simulink model "Partie6_RRC"  (R2026b)
settings: Solver=FixedStepDiscrete  StopTime=Nbits*Tb  FixedStep=Tf
undefined symbols (not defined in the file): D_ech, graine, graine_bruit, h_rx, h_tx, p1, Tb, Te, variance_bruit_p6
libraries: simulink x2, dspsigops x1
settings Model: Creator=WORLD COMPUTERS  LastModifiedBy=WORLD COMPUTERS

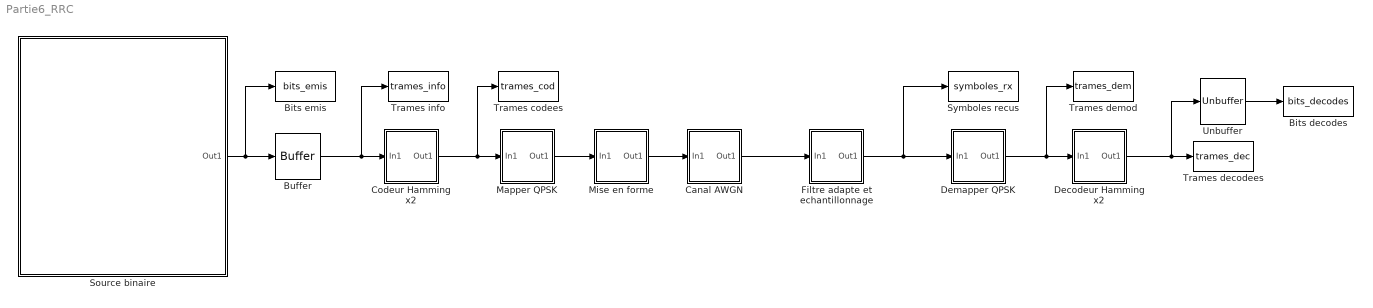
== system Partie6_RRC ==
  Bits decodes : ToWorkspace  VariableName=bits_decodes  SampleTime=-1
  Bits emis : ToWorkspace  VariableName=bits_emis  SampleTime=-1
  Buffer : Buffer  N=8
  Canal AWGN : Subsystem
  Codeur Hamming x2 : Subsystem
  Decodeur Hamming x2 : Subsystem
  Demapper QPSK : Subsystem
  Filtre adapte et echantillonnage : Subsystem
  Mapper QPSK : Subsystem
  Mise en forme : Subsystem
  Source binaire : Subsystem
  Symboles recus : ToWorkspace  VariableName=symboles_rx  SampleTime=-1
  Trames codees : ToWorkspace  VariableName=trames_cod  SampleTime=-1
  Trames decodees : ToWorkspace  VariableName=trames_dec  SampleTime=-1
  Trames demod : ToWorkspace  VariableName=trames_dem  SampleTime=-1
  Trames info : ToWorkspace  VariableName=trames_info  SampleTime=-1
  Unbuffer : Unbuffer
  wires:
  Source binaire/1(Out1) -> Buffer/1, Bits emis/1
  Demapper QPSK/1(Out1) -> Trames demod/1, Decodeur Hamming x2/1(In1)
  Buffer/1 -> Codeur Hamming x2/1(In1), Trames info/1
  Codeur Hamming x2/1(Out1) -> Mapper QPSK/1(In1), Trames codees/1
  Mapper QPSK/1(Out1) -> Mise en forme/1(In1)
  Mise en forme/1(Out1) -> Canal AWGN/1(In1)
  Filtre adapte et echantillonnage/1(Out1) -> Demapper QPSK/1(In1), Symboles recus/1
  Canal AWGN/1(Out1) -> Filtre adapte et echantillonnage/1(In1)
  Decodeur Hamming x2/1(Out1) -> Unbuffer/1, Trames decodees/1
  Unbuffer/1 -> Bits decodes/1

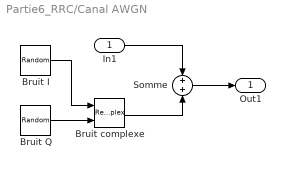
== system Partie6_RRC/Canal AWGN ==
  In1 : Inport
  Bruit I : RandomNumber  Variance=variance_bruit_p6  Seed=graine_bruit  SampleTime=Te
  Bruit Q : RandomNumber  Variance=variance_bruit_p6  Seed=graine_bruit+100  SampleTime=Te
  Bruit complexe : RealImagToComplex
  Somme : Sum
  Out1 : Outport
  wires:
  Bruit I/1 -> Bruit complexe/1
  Bruit complexe/1 -> Somme/2
  In1/1 -> Somme/1
  Bruit Q/1 -> Bruit complexe/2
  Somme/1 -> Out1/1

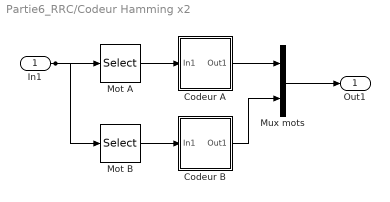
== system Partie6_RRC/Codeur Hamming x2 ==
  In1 : Inport
  Codeur A : Subsystem
  Codeur B : Subsystem
  Mot A : Selector  InputPortWidth=8  IndexOptions=Index vector (dialog)  Indices=[1 2 3 4]  OutputSizes=1
  Mot B : Selector  InputPortWidth=8  IndexOptions=Index vector (dialog)  Indices=[5 6 7 8]  OutputSizes=1
  Mux mots : Mux  Inputs=2
  Out1 : Outport
  wires:
  Mot B/1 -> Codeur B/1(In1)
  In1/1 -> Mot A/1, Mot B/1
  Codeur A/1(Out1) -> Mux mots/1
  Mot A/1 -> Codeur A/1(In1)
  Codeur B/1(Out1) -> Mux mots/2
  Mux mots/1 -> Out1/1

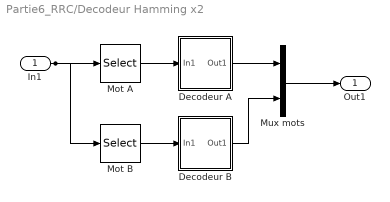
== system Partie6_RRC/Decodeur Hamming x2 ==
  In1 : Inport
  Decodeur A : Subsystem
  Decodeur B : Subsystem
  Mot A : Selector  InputPortWidth=14  IndexOptions=Index vector (dialog)  Indices=[1 2 3 4 5 6 7]  OutputSizes=1
  Mot B : Selector  InputPortWidth=14  IndexOptions=Index vector (dialog)  Indices=[8 9 10 11 12 13 14]  OutputSizes=1
  Mux mots : Mux  Inputs=2
  Out1 : Outport
  wires:
  Mot B/1 -> Decodeur B/1(In1)
  In1/1 -> Mot A/1, Mot B/1
  Mot A/1 -> Decodeur A/1(In1)
  Decodeur A/1(Out1) -> Mux mots/1
  Decodeur B/1(Out1) -> Mux mots/2
  Mux mots/1 -> Out1/1

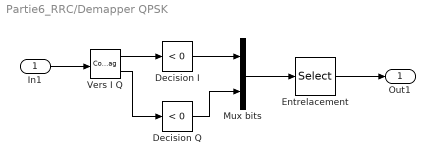
== system Partie6_RRC/Demapper QPSK ==
  In1 : Inport
  Decision I : simulink/Logic and Bit Operations/Compare To Constant  relop=<  const=0  OutDataTypeStr=boolean
  Decision Q : simulink/Logic and Bit Operations/Compare To Constant  relop=<  const=0  OutDataTypeStr=boolean
  Entrelacement : Selector  InputPortWidth=14  IndexOptions=Index vector (dialog)  Indices="[1   8   2   9   3  10   4  11   5  12   6  13   7  14]"  OutputSizes=1
  Mux bits : Mux  Inputs=2
  Vers I Q : ComplexToRealImag
  Out1 : Outport
  wires:
  Entrelacement/1 -> Out1/1
  In1/1 -> Vers I Q/1
  Mux bits/1 -> Entrelacement/1
  Decision Q/1 -> Mux bits/2
  Vers I Q/1 -> Decision I/1
  Vers I Q/2 -> Decision Q/1
  Decision I/1 -> Mux bits/1

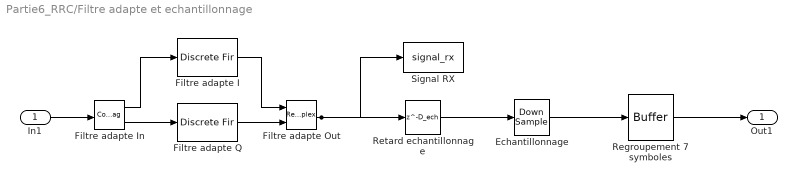
== system Partie6_RRC/Filtre adapte et echantillonnage ==
  In1 : Inport
  Echantillonnage : DownSample  DownsamplingFactor=L  RateOptions=Allow multirate processing  AllowArbitraryFixedInput=on
  Filtre adapte I : DiscreteFir  Coefficients=h_rx
  Filtre adapte In : ComplexToRealImag
  Filtre adapte Out : RealImagToComplex
  Filtre adapte Q : DiscreteFir  Coefficients=h_rx
  Regroupement 7 symboles : Buffer  N=7
  Retard echantillonnage : Delay  DelayLength=D_ech  InitialCondition=0
  Signal RX : ToWorkspace  VariableName=signal_rx  SampleTime=-1
  Out1 : Outport
  wires:
  Echantillonnage/1 -> Regroupement 7 symboles/1
  Retard echantillonnage/1 -> Echantillonnage/1
  Filtre adapte Out/1 -> Retard echantillonnage/1, Signal RX/1
  In1/1 -> Filtre adapte In/1
  Filtre adapte Q/1 -> Filtre adapte Out/2
  Filtre adapte I/1 -> Filtre adapte Out/1
  Filtre adapte In/2 -> Filtre adapte Q/1
  Filtre adapte In/1 -> Filtre adapte I/1
  Regroupement 7 symboles/1 -> Out1/1

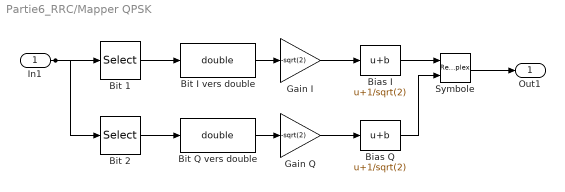
== system Partie6_RRC/Mapper QPSK ==
  In1 : Inport
  Bias I : Bias  Bias=1/sqrt(2)  SaturateOnIntegerOverflow=off
  Bias Q : Bias  Bias=1/sqrt(2)  SaturateOnIntegerOverflow=off
  Bit 1 : Selector  InputPortWidth=14  IndexOptions=Index vector (dialog)  Indices="[1   3   5   7   9  11  13]"  OutputSizes=1
  Bit 2 : Selector  InputPortWidth=14  IndexOptions=Index vector (dialog)  Indices="[2   4   6   8  10  12  14]"  OutputSizes=1
  Bit I vers double : DataTypeConversion  OutDataTypeStr=double  SaturateOnIntegerOverflow=off  RndMeth=Floor
  Bit Q vers double : DataTypeConversion  OutDataTypeStr=double  SaturateOnIntegerOverflow=off  RndMeth=Floor
  Gain I : Gain  Gain=-sqrt(2)
  Gain Q : Gain  Gain=-sqrt(2)
  Symbole : RealImagToComplex
  Out1 : Outport
  wires:
  In1/1 -> Bit 1/1, Bit 2/1
  Gain I/1 -> Bias I/1
  Bit I vers double/1 -> Gain I/1
  Bit Q vers double/1 -> Gain Q/1
  Bit 2/1 -> Bit Q vers double/1
  Bit 1/1 -> Bit I vers double/1
  Bias I/1 -> Symbole/1
  Gain Q/1 -> Bias Q/1
  Bias Q/1 -> Symbole/2
  Symbole/1 -> Out1/1

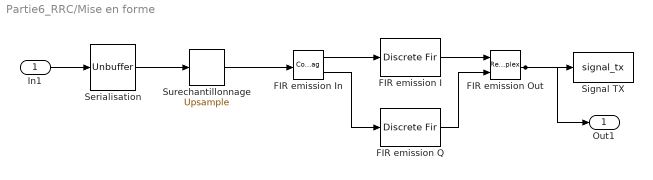
== system Partie6_RRC/Mise en forme ==
  In1 : Inport
  FIR emission I : DiscreteFir  Coefficients=h_tx
  FIR emission In : ComplexToRealImag
  FIR emission Out : RealImagToComplex
  FIR emission Q : DiscreteFir  Coefficients=h_tx
  Serialisation : Unbuffer
  Signal TX : ToWorkspace  VariableName=signal_tx  SampleTime=-1
  Surechantillonnage : dspsigops/Upsample  FactorSource=Dialog parameter  UpsamplingFactor=L  MaxUpsamplingFactor=16  SampleOffset=0  RateOptions=Allow multirate processing  InitialConditions=0  mode=Unused parameter value
  Out1 : Outport
  wires:
  Serialisation/1 -> Surechantillonnage/1
  In1/1 -> Serialisation/1
  FIR emission Out/1 -> Out1/1, Signal TX/1
  Surechantillonnage/1 -> FIR emission In/1
  FIR emission In/2 -> FIR emission Q/1
  FIR emission In/1 -> FIR emission I/1
  FIR emission Q/1 -> FIR emission Out/2
  FIR emission I/1 -> FIR emission Out/1

== system Partie6_RRC/Source binaire ==
  Constant : Constant  Value=p1
  Relational Operator : RelationalOperator  Operator=<  OutDataTypeStr=boolean  RndMeth=Simplest  InputSameDT=off
  Uniform Random Number : UniformRandomNumber  Minimum=0  Seed=graine  SampleTime=Tb
  Out1 : Outport
  wires:
  Relational Operator/1 -> Out1/1
  Constant/1 -> Relational Operator/2
  Uniform Random Number/1 -> Relational Operator/1

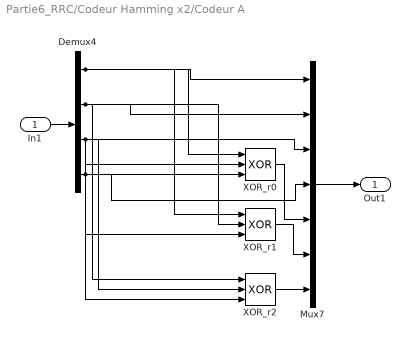
== system Partie6_RRC/Codeur Hamming x2/Codeur A ==
  In1 : Inport
  Demux4 : Demux
  Mux7 : Mux  Inputs=7
  XOR_r0 : Logic  Operator=XOR  Inputs=3  AllPortsSameDT=off  OutDataTypeStr=boolean
  XOR_r1 : Logic  Operator=XOR  Inputs=3  AllPortsSameDT=off  OutDataTypeStr=boolean
  XOR_r2 : Logic  Operator=XOR  Inputs=3  AllPortsSameDT=off  OutDataTypeStr=boolean
  Out1 : Outport
  wires:
  Mux7/1 -> Out1/1
  XOR_r1/1 -> Mux7/6
  XOR_r2/1 -> Mux7/7
  XOR_r0/1 -> Mux7/5
  Demux4/1 -> XOR_r1/1, XOR_r0/1, Mux7/1
  Demux4/2 -> XOR_r2/1, XOR_r1/2, Mux7/2
  Demux4/3 -> XOR_r2/2, XOR_r1/3, XOR_r0/2, Mux7/3
  Demux4/4 -> XOR_r2/3, XOR_r0/3, Mux7/4
  In1/1 -> Demux4/1

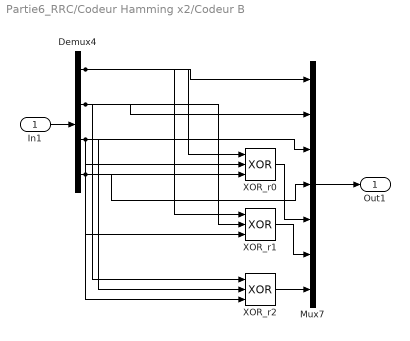
== system Partie6_RRC/Codeur Hamming x2/Codeur B ==
  In1 : Inport
  Demux4 : Demux
  Mux7 : Mux  Inputs=7
  XOR_r0 : Logic  Operator=XOR  Inputs=3  AllPortsSameDT=off  OutDataTypeStr=boolean
  XOR_r1 : Logic  Operator=XOR  Inputs=3  AllPortsSameDT=off  OutDataTypeStr=boolean
  XOR_r2 : Logic  Operator=XOR  Inputs=3  AllPortsSameDT=off  OutDataTypeStr=boolean
  Out1 : Outport
  wires:
  Mux7/1 -> Out1/1
  XOR_r1/1 -> Mux7/6
  XOR_r2/1 -> Mux7/7
  XOR_r0/1 -> Mux7/5
  Demux4/1 -> XOR_r1/1, XOR_r0/1, Mux7/1
  Demux4/2 -> XOR_r2/1, XOR_r1/2, Mux7/2
  Demux4/3 -> XOR_r2/2, XOR_r1/3, XOR_r0/2, Mux7/3
  Demux4/4 -> XOR_r2/3, XOR_r0/3, Mux7/4
  In1/1 -> Demux4/1

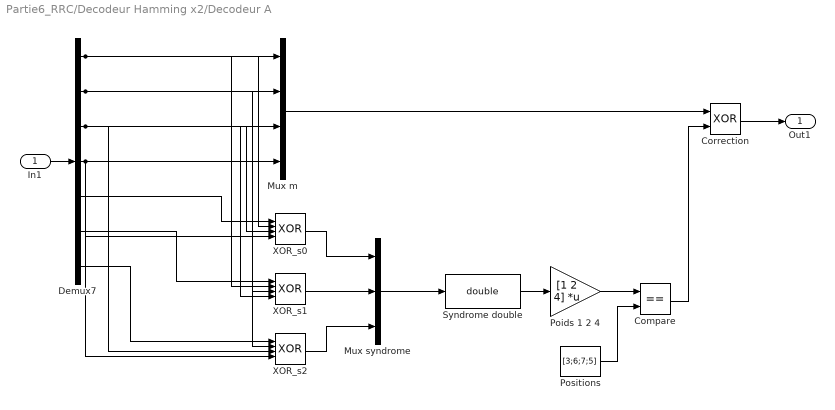
== system Partie6_RRC/Decodeur Hamming x2/Decodeur A ==
  In1 : Inport
  Compare : RelationalOperator  Operator===  OutDataTypeStr=boolean  RndMeth=Simplest  InputSameDT=off
  Correction : Logic  Operator=XOR  AllPortsSameDT=off  OutDataTypeStr=boolean
  Demux7 : Demux  Outputs=7
  Mux m : Mux
  Mux syndrome : Mux  Inputs=3
  Poids 1 2 4 : Gain  Gain=[1 2 4]  Multiplication=Matrix(K*u)
  Positions : Constant  Value=[3;6;7;5]
  Syndrome double : DataTypeConversion  OutDataTypeStr=double  SaturateOnIntegerOverflow=off  RndMeth=Floor
  XOR_s0 : Logic  Operator=XOR  Inputs=4  AllPortsSameDT=off  OutDataTypeStr=boolean
  XOR_s1 : Logic  Operator=XOR  Inputs=4  AllPortsSameDT=off  OutDataTypeStr=boolean
  XOR_s2 : Logic  Operator=XOR  Inputs=4  AllPortsSameDT=off  OutDataTypeStr=boolean
  Out1 : Outport
  wires:
  Correction/1 -> Out1/1
  Positions/1 -> Compare/2
  Compare/1 -> Correction/2
  Syndrome double/1 -> Poids 1 2 4/1
  Mux m/1 -> Correction/1
  Poids 1 2 4/1 -> Compare/1
  Demux7/1 -> Mux m/1, XOR_s1/2, XOR_s0/2
  XOR_s1/1 -> Mux syndrome/2
  Demux7/2 -> Mux m/2, XOR_s2/2, XOR_s1/3
  Demux7/3 -> Mux m/3, XOR_s2/3, XOR_s1/4, XOR_s0/3
  XOR_s0/1 -> Mux syndrome/1
  Demux7/4 -> Mux m/4, XOR_s2/4, XOR_s0/4
  Demux7/5 -> XOR_s0/1
  Mux syndrome/1 -> Syndrome double/1
  Demux7/6 -> XOR_s1/1
  Demux7/7 -> XOR_s2/1
  XOR_s2/1 -> Mux syndrome/3
  In1/1 -> Demux7/1

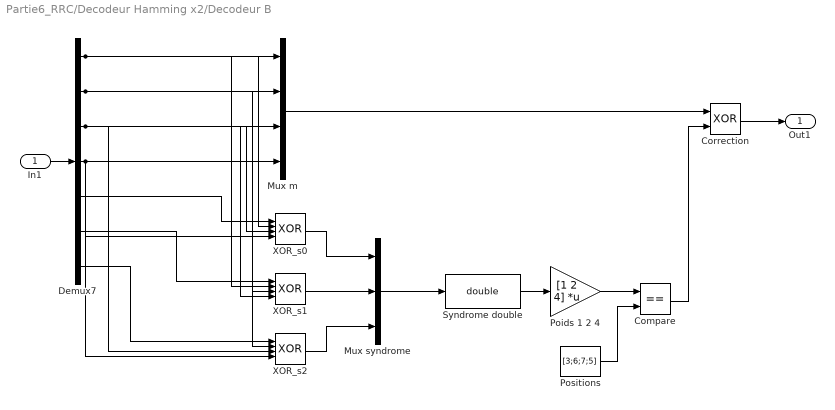
== system Partie6_RRC/Decodeur Hamming x2/Decodeur B ==
  In1 : Inport
  Compare : RelationalOperator  Operator===  OutDataTypeStr=boolean  RndMeth=Simplest  InputSameDT=off
  Correction : Logic  Operator=XOR  AllPortsSameDT=off  OutDataTypeStr=boolean
  Demux7 : Demux  Outputs=7
  Mux m : Mux
  Mux syndrome : Mux  Inputs=3
  Poids 1 2 4 : Gain  Gain=[1 2 4]  Multiplication=Matrix(K*u)
  Positions : Constant  Value=[3;6;7;5]
  Syndrome double : DataTypeConversion  OutDataTypeStr=double  SaturateOnIntegerOverflow=off  RndMeth=Floor
  XOR_s0 : Logic  Operator=XOR  Inputs=4  AllPortsSameDT=off  OutDataTypeStr=boolean
  XOR_s1 : Logic  Operator=XOR  Inputs=4  AllPortsSameDT=off  OutDataTypeStr=boolean
  XOR_s2 : Logic  Operator=XOR  Inputs=4  AllPortsSameDT=off  OutDataTypeStr=boolean
  Out1 : Outport
  wires:
  Correction/1 -> Out1/1
  Positions/1 -> Compare/2
  Compare/1 -> Correction/2
  Syndrome double/1 -> Poids 1 2 4/1
  Mux m/1 -> Correction/1
  Poids 1 2 4/1 -> Compare/1
  Demux7/1 -> Mux m/1, XOR_s1/2, XOR_s0/2
  XOR_s1/1 -> Mux syndrome/2
  Demux7/2 -> Mux m/2, XOR_s2/2, XOR_s1/3
  Demux7/3 -> Mux m/3, XOR_s2/3, XOR_s1/4, XOR_s0/3
  XOR_s0/1 -> Mux syndrome/1
  Demux7/4 -> Mux m/4, XOR_s2/4, XOR_s0/4
  Demux7/5 -> XOR_s0/1
  Mux syndrome/1 -> Syndrome double/1
  Demux7/6 -> XOR_s1/1
  Demux7/7 -> XOR_s2/1
  XOR_s2/1 -> Mux syndrome/3
  In1/1 -> Demux7/1
